simulink model "BMS_UV_Protection_Test"  (R2025b)
settings: Solver=FixedStepDiscrete  StartTime=0.0  StopTime=6  FixedStep=Ts  RelTol=1e-3
undefined symbols (not defined in the file): Ts
settings Model: Creator=Khadija  LastModifiedBy=Khadija

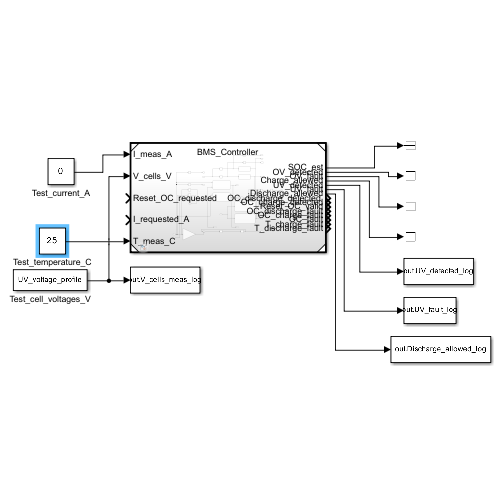
[thumbnail: Simulink's stored preview of the top-level diagram]
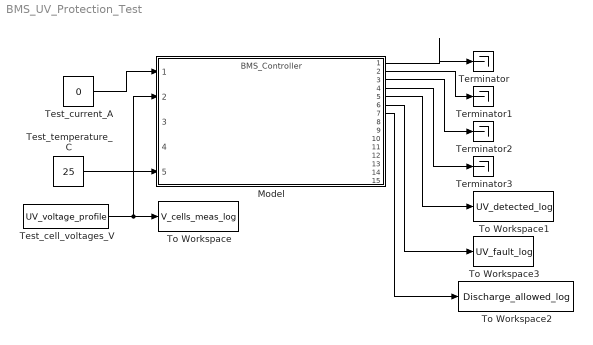
== system BMS_UV_Protection_Test ==
  Model : ModelReference  ModelNameDialog=BMS_Controller  SimulationMode=Normal  ModelReferenceVersion=1.40
  Terminator{,1..3} (4 alike) : Terminator
  Test_cell_voltages_V : FromWorkspace  VariableName=UV_voltage_profile  SampleTime=Ts  Interpolate=off  ZeroCross=off  OutputAfterFinalValue=Holding final value
  Test_current_A : Constant  Value=0  SampleTime=Ts
  Test_temperature_C : Constant  Value=25  OutDataTypeStr=double  SampleTime=Ts
  To Workspace : ToWorkspace  VariableName=V_cells_meas_log  SaveFormat=Timeseries  SampleTime=-1
  To Workspace1 : ToWorkspace  VariableName=UV_detected_log  SaveFormat=Timeseries  SampleTime=-1
  To Workspace2 : ToWorkspace  VariableName=Discharge_allowed_log  SaveFormat=Timeseries  SampleTime=-1
  To Workspace3 : ToWorkspace  VariableName=UV_fault_log  SaveFormat=Timeseries  SampleTime=-1
  wires:
  Model/3 -> Terminator2/1
  Model/2 -> Terminator1/1
  Model/1 -> Terminator/1
  Test_cell_voltages_V/1 -> Model/2, To Workspace/1
  Test_current_A/1 -> Model/1
  Model/4 -> Terminator3/1
  Model/6 -> To Workspace3/1
  Model/5 -> To Workspace1/1
  Model/7 -> To Workspace2/1
  Test_temperature_C/1 -> Model/5
